simulink model "sf_slscheduler"  (R2025b)
settings: Solver=FixedStepDiscrete  StartTime=0.0  StopTime=10.0  FixedStep=0.01  RelTol=1e-3  EnableMultiTasking=on
settings Model: Creator=The MathWorks, Inc.  LastModifiedBy=The MathWorks, Inc.
settings SolverCC: AlgebraicLoopSolver=TrustRegion
settings DataIOCC: LimitDataPoints=on  SaveFormat=Array  ReturnWorkspaceOutputs=off
settings OptimizationCC: ReuseModelBlockBuffer=off  ExpressionDepthLimit=2147483647.0  LifeSpan=inf
settings DebuggingCC: UnderspecifiedInitializationDetection=Classic  MergeDetectMultiDrivingBlocksExec=none  SolverPrmCheckMsg=warning  FcnCallInpInsideContextMsg=warning  UnconnectedInputMsg=warning  UnconnectedOutputMsg=warning  UnconnectedLineMsg=warning  StateNameClashWarn=warning  SFUnexpectedBacktrackingDiag=warning  SFNoUnconditionalDefaultTransitionDiag=warning  SFExecutionAtInitializationDiag=none  ArithmeticOperatorsInVariantConditions=warning
settings HardwareCC: ProdBitPerPointer=32.0  ProdBitPerSizeT=32.0  ProdBitPerPtrDiffT=32.0  ProdLargestAtomicFloat=None  ProdIntDivRoundTo=Undefined  ProdEndianess=Unspecified  ProdWordSize=32.0  ProdHWDeviceType=32-bit Generic
settings ModelReferenceCC: EnableRefExpFcnMdlSchedulingChecks=on  PropagateSignalLabelsOutOfModel=off
settings SFSimCC: SimUseLocalCustomCode=off  SimParseCustomCode=off  CustomCodeUndefinedFunction=UseInterfaceOnly
settings RTWCC: RTWUseLocalCustomCode=off  GPUComputeCapability=3.5
settings CodeAppCC: StateflowObjectComments=on
settings GRTTargetCC: TargetLangStandard=C89/C90 (ANSI)  CombineOutputUpdateFcns=off  GRTInterface=on
settings ConfigComp: CovMetricSettings=dw  CovSaveCumulativeToWorkspaceVar=on  CovSaveSingleToWorkspaceVar=on  CovExternalEMLEnable=off  CovSFcnEnable=off

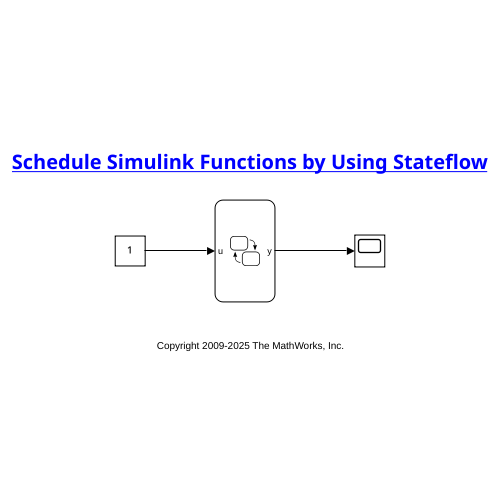
[thumbnail: Simulink's stored preview of the top-level diagram]
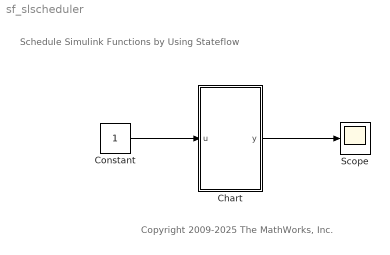
== system sf_slscheduler ==
  note: Copyright 2009-2025 The MathWorks, Inc.
  note: Schedule Simulink Functions by Using Stateflow
  Chart : Stateflow chart  TreatAsAtomicUnit=on
  Constant : Constant
  Scope : Scope
      settings: ActiveDisplayYMinimum=0  ActiveDisplayYMaximum=350
  wires:
  Chart/1(y) -> Scope/1
  Constant/1 -> Chart/1(u)

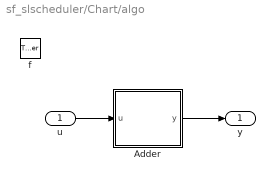
== system sf_slscheduler/Chart/algo ==
  u : Inport
  f : TriggerPort  TriggerType=function-call  VariantControl=(inherit)
      settings: CopyFcn=Stateflow.SLINSF.SimulinkMan.removeBlockPreDeleteFcn  PreDeleteFcn=Stateflow.SLINSF.SimulinkMan.unsafePredeleteFcn
  Adder : Subsystem
  y : Outport  VectorParamsAs1DForOutWhenUnconnected=off
  wires:
  u/1 -> Adder/1(u)
  Adder/1(y) -> y/1

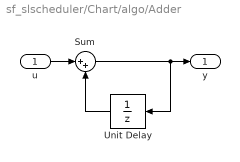
== system sf_slscheduler/Chart/algo/Adder ==
  u : Inport
  Sum : Sum  Inputs=|++
  Unit Delay : UnitDelay  SampleTime=-1  HasFrameUpgradeWarning=on
  y : Outport  VectorParamsAs1DForOutWhenUnconnected=off
  wires:
  Sum/1 -> Unit Delay/1, y/1
  Unit Delay/1 -> Sum/2
  u/1 -> Sum/1

== stateflow chart sf_slscheduler/Chart ==
  state Fast_Scheduler
    on every(2,tick): y = algo(u);
  state Slow_Scheduler
    on every(5,tick): y = algo(u);
  state y = algo(u) [function]
  (default) -> Fast_Scheduler
  Fast_Scheduler -> Slow_Scheduler : after(1.5,sec)
  Slow_Scheduler -> Fast_Scheduler : after(3.5,sec)
  data: u function_input; y function_output; u input; y output double
